simulink model "interleaved_boost_compact"  (R2026b)
settings: Solver=ode23tb  StopTime=param.sim.simlength  MaxStep=param.glb_time.tc
values from neighbouring files (symbols this model uses):
  param = struct()    [init_model.m]
libraries: fl_lib x2, nesl_utility x1, lithium_ion_battery x1, interleaved_boost_3legs x1
settings Model: Creator=d.bagnara  LastModifiedBy=d.bagnara
settings SolverCC: ZeroCrossControl=DisableAll
settings DataIOCC: SaveOutput=off  SaveTime=off
settings SimscapeCC: SimscapeNominalValues="[{\"value\":\"1\",\"unit\":\"A\"},{\"value\":\"1\",\"unit\":\"bar\"},{\"value\":\"1\",\"unit\":\"cm^2\"},{\"value\":\"1\",\"unit\":\"cm^3/s\"},{\"value\":\"1\",\"unit\":\"kJ/kg\"},{\"value\":\"1\",\"unit\":\"kW\"},{\"value\":\"1\",\"unit\":\"l\"},{\"value\":\"1\",\"unit\":\"N\"},{\"value\":\"1\",\"unit\":\"N*m\"},{\"value\":\"1\",\"unit\":\"V\"},{\"value\":\"0.001\",\"unit\":\"Wb\"}]"  SimscapeUseEnergyAccounting=off

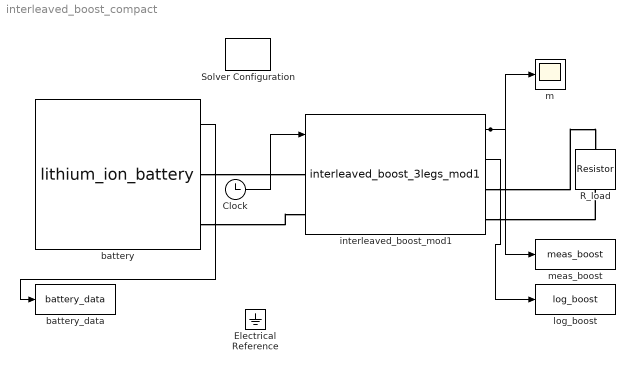
== system interleaved_boost_compact ==
  Clock : Clock
  Electrical Reference : fl_lib/Electrical/Electrical Elements/Electrical Reference
  R_load : fl_lib/Electrical/Electrical Elements/Resistor  R=param.load.R_load Ohm  i_specify=off  i_priority=None  i=0 A  i_nominal_specify=off  i_nominal_value=1  i_nominal_unit=A  v_specify=off  v_priority=None  v=0 V  v_nominal_specify=off  v_nominal_value=1  v_nominal_unit=V
  Solver Configuration : nesl_utility/Solver Configuration  PhysicalDomain=network_engine_domain  SubClassName=solver  LeftPortType=input  RightPortType=generic  Tones=[]  Harmonics=[]  SimulateNoise=off  Profile=off  UseLocalSampling=off  EnableSwitchedLinearOptims=on  FrequencyDomain=off  UseCCode=off  RelTol=0.001  AbsTol=0.001  MinStep=1e-09  ToWorkspace=off  RevertToSquareIcSolve=off  NumHomotopyIterations=100  PhasorMode=off  PhasorModeNumHarmonics=1  ConsistencySolver=NEWTON_XTOL_AFTER_FTOL  CanonicalOrdering=CANONICAL  OptimizeIntermediates=OPTIMIZED  MulticoreSolverChoice=BACKWARD_EULER  IndexReductionMethod=DerivativeReplacement  DoDC=off  ResidualTolerance=1e-09  ConsistencyTolSource=GLOBAL  ConsistencyAbsTol=0.001  ConsistencyRelTol=0.001  ConsistencyTolFactor=0.001  UseLocalSolver=on  LocalSolverChoice=NE_BACKWARD_EULER_ADVANCER  ResolveIndetEquations=on  FunctionEvalNumThread=1  LocalSolverSampleTime=param.glb_time.tc  DoFixedCost=on  MaxNonlinIter=param.sim.nonlinear_iterations  MaxModeIter=2  ComputeImpulses=off  ImpulseIterations=2  LinearAlgebra=auto  LinearAlgebraNumThread=0  EquationFormulation=NE_TIME_EF  DelaysMemoryBudget=1024  AutomaticFiltering=on  FilteringTimeConstant=0.001  PartitionStorageMethod=AS_NEEDED  PartitionMemoryBudget=1024  PartitionMethod=BALANCED  MultibodyUseLocalSolver=off  MultibodyLocalSolverChoice=ODE1  MultibodyLocalSolverSampleTime=0.001
  battery : lithium_ion_battery/lithium_ion_battery  Q=param.battery.pack_1.Q  number_of_cells=param.battery.pack_1.number_of_cells  E_1=param.battery.pack_1.E_1  E0=param.battery.pack_1.E0  E1=param.battery.pack_1.E1  E2=param.battery.pack_1.E2  E3=param.battery.pack_1.E3  Elog=param.battery.pack_1.Elog  R0=param.battery.pack_1.R0  R1=param.battery.pack_1.R1  C1=param.battery.pack_1.C1  M=param.battery.pack_1.M  alpha=param.battery.pack_1.alpha  soc_init=param.battery.pack_1.soc_init  ts_battery=param.glb_time.ts_dab  q1Kalman=param.battery.pack_1.q1Kalman  q2Kalman=param.battery.pack_1.q2Kalman  q3Kalman=param.battery.pack_1.q3Kalman  rKalman=param.battery.pack_1.rKalman  tc=param.glb_time.tc  enable_white_noise_m=0  battery_voltage_init_m=param.battery.nominal_battery_voltage_1
  battery_data : ToWorkspace  VariableName=battery_data  SaveFormat=Timeseries  SampleTime=param.glb_time.tc
      settings: Decimation=param.glb_time.decimation_tc
  interleaved_boost_mod1 : interleaved_boost_3legs/interleaved_boost_3legs_mod1  p=param.boost
  log_boost : ToWorkspace  VariableName=log_boost  SaveFormat=Timeseries  SampleTime=param.glb_time.tc
      settings: Decimation=param.glb_time.decimation_tc
  m : Scope
  meas_boost : ToWorkspace  VariableName=meas_boost  SaveFormat=Timeseries  SampleTime=param.glb_time.tc
      settings: Decimation=param.glb_time.decimation_tc
  wires:
  Clock/1 -> interleaved_boost_mod1/1
  interleaved_boost_mod1/1 -> meas_boost/1, m/1
  interleaved_boost_mod1/2 -> log_boost/1
  battery/1 -> battery_data/1
  connections:
  battery/RConn1 -- interleaved_boost_mod1/LConn1
  battery/RConn2 -- interleaved_boost_mod1/LConn2
  interleaved_boost_mod1/RConn1 -- R_load/LConn1
  interleaved_boost_mod1/RConn2 -- R_load/RConn1
